simulink model "ac1_op_unlinked_R2016a"  (R2016a)
settings: Solver=ode23tb  SolverMode=SingleTasking  StartTime=0.0  StopTime=5  RelTol=1e-4
InitFcn:
  | %% Sys Para
  | fsw=10e3;
  | Ts_Control=1/fsw;
  | Tscon=Ts_Control;
  | Ts_Power=Ts_Control/32;
undefined symbols (not defined in the file): L2, R1, Rd
libraries: powerlib x8, powerlib_meascontrol x5
Description:
  | Copyright 2008-2017 The MathWorks, Inc.
settings Model: ExtModeTrigMode=oneshot  ExtModeArmWhenConnect=off  ExtModeAutoUpdateStatusClock=off  Creator=MathWorks  LastModifiedBy=CXIE
settings DataIOCC: ExternalInput=[]  SaveFormat=Array  SignalLoggingSaveFormat=ModelDataLogs  SaveOutput=off  SaveTime=off  SignalLoggingName=sigsOut
settings OptimizationCC: BlockReduction=off  BooleanDataType=off  ExpressionDepthLimit=2147483647  InitFltsAndDblsToZero=on  EfficientMapNaN2IntZero=off
settings DebuggingCC: UnderspecifiedInitializationDetection=Classic  MergeDetectMultiDrivingBlocksExec=none  CheckExecutionContextPreStartOutputMsg=on  CheckExecutionContextRuntimeOutputMsg=on  SignalResolutionControl=TryResolveAllWithWarning  MultiTaskDSMMsg=warning  MultiTaskCondExecSysMsg=none  SigSpecEnsureSampleTimeMsg=none  FcnCallInpInsideContextMsg=EnableAllAsWarning  StateNameClashWarn=warning
settings HardwareCC: ProdBitPerPointer=32  ProdLargestAtomicFloat=None  ProdIntDivRoundTo=Undefined  ProdEndianess=Unspecified  ProdWordSize=32  ProdHWDeviceType=32-bit Generic  TargetUnknown=on
settings ModelReferenceCC: PropagateSignalLabelsOutOfModel=off
settings GRTTargetCC: CombineOutputUpdateFcns=off  GRTInterface=on
settings ConfigComp: CovSFcnEnable=off
settings SimscapeCC: SimscapeNormalizeSystem=off  SimscapeNominalValues={1, 'bar'; 1, 'cm^3/s'; 1, 'bar*kg/s'; 1, 'kJ/kg'; 1, 'kW'; }

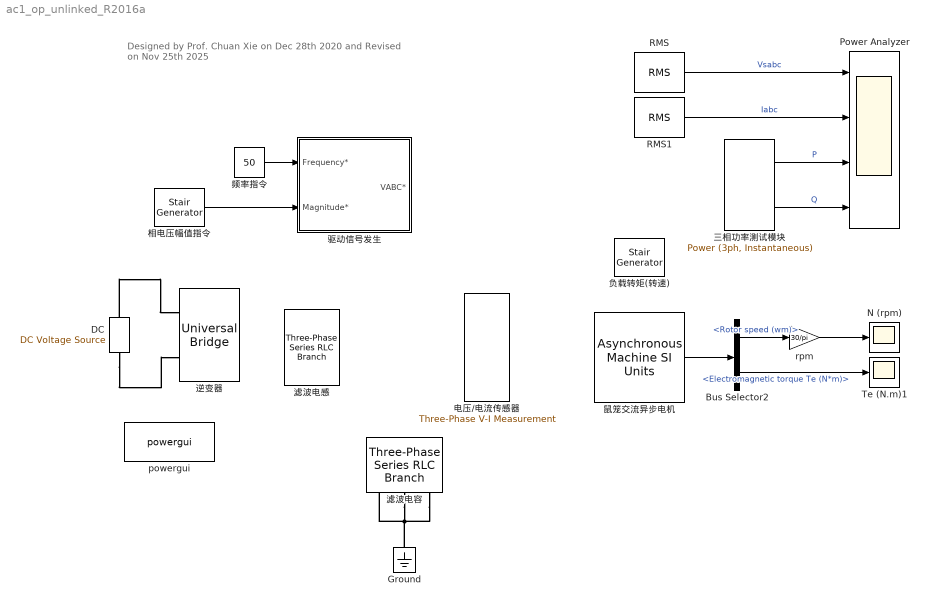
== system ac1_op_unlinked_R2016a ==
  note: Designed by Prof. Chuan Xie
      | on Dec 28th 2020
      | and Revised on Nov 25th 2025
  Bus Selector2 : BusSelector  OutputSignals=Mechanical.Rotor speed (wm),Mechanical.Electromagnetic torque Te (N*m)
  DC : powerlib/Electrical Sources/DC Voltage Source  Amplitude=650  Measurements=None
  Ground : powerlib/Elements/Ground  LConnTagsString=a
  N (rpm) : Scope
  Power Analyzer : Scope  NumInputPorts=4
  RMS : powerlib_meascontrol/Measurements/RMS  TrueRMS=on  Freq=50  RMSInit=120  Ts=0
  RMS1 : powerlib_meascontrol/Measurements/RMS  TrueRMS=on  Freq=50  RMSInit=120  Ts=0
  Te (N.m)1 : Scope
  powergui : powerlib/powergui  SimulationMode=Continuous  SampleTime=Ts_Power  frequency=60  Iterations=50  frequencyindice=50  Pbase=100e6  ErrMax=1e-4  UnitsV=kV  UnitsW=MW  buscounter=0  FunctionMessages=off  echomessages=off  EnableUseOfTLC=off  CurrentSourceSwitches=off  DisableSnubberDevices=off  DisableRonSwitches=off  DisableVfSwitches=off  DisplayEquations=off  AutomaticDiscreteSolvers=off  SolverType=Tustin  Interpol=off  ExternalGateDelay=off  methode=off  Ts=0  x0status=blocks  SPID=on  SwTol=0  HookPort=off  NonlinearTolerance=1e-4  nMaxIteration=100  ContinueOnMaxIteration=off  RestoreLinks=warning  ResistiveCurrentMeasurement=off  Frange=[0:2:500]  Ylog=off  Xlog=on  ShowGrid=off  save=off  variable=ZData  structure=0  ZoomFFT=on  StartTime=0.0  cycles=1  DisplayStyle=1  fundamental=60  FreqAxis=off  MaxFrequency=1000  frequencyindicesteady=1  RmsSteady=1  display=off
  rpm : Gain  Gain=30/pi  SaturateOnIntegerOverflow=on  OutDataTypeStr=Inherit: Same as input  ParamDataTypeStr=Inherit: Same as input
  三相功率测试模块 : powerlib_meascontrol/Measurements/Power (3ph, Instantaneous)
  滤波电容 : powerlib/Elements/Three-Phase Series RLC Branch  LConnTagsString=A|B|C  RConnTagsString=A|B|C  BranchType=C  Resistance=Rd  Inductance=L2  Capacitance=10e-6  Measurements=Branch currents
  滤波电感 : powerlib/Elements/Three-Phase Series RLC Branch  LConnTagsString=A|B|C  RConnTagsString=A|B|C  BranchType=L  Resistance=R1  Inductance=1e-3  Capacitance=1e-6  Measurements=Branch currents
  电压/电流传感器 : powerlib/Measurements/Three-Phase V-I Measurement  VoltageMeasurement=phase-to-ground  SetLabelV=off  LabelV=Vc1  Vpu=off  VpuLL=off  CurrentMeasurement=yes  SetLabelI=off  LabelI=IL1  Ipu=off  Pbase=100e6  Vbase=280  OutputType=Complex  PhasorSimulation=off  PSBequivalent=0
  相电压幅值指令 : powerlib_meascontrol/Pulse & Signal Generators/Stair Generator  t=[0]  e=[0]  Ts=0
  负载转矩(转速) : powerlib_meascontrol/Pulse & Signal Generators/Stair Generator  t=[0]  e=[0]  Ts=0
  逆变器 : powerlib/Power Electronics/Universal Bridge  Arms=3  SnubberResistance=1e5  SnubberCapacitance=inf  Device=Average-model based VSC  Ron=1e-3  Lon=0  ForwardVoltages="[  0  0  ]"  ForwardVoltage=0  GTOparameters=[ 10e-6 , 20e-6 ]  IGBTparameters=[ 1e-6 , 2e-6 ]  Measurements=None  Measurements_2=None  converterType=Rectifier
  频率指令 : Constant  Value=50
  驱动信号发生 : Subsystem
  鼠笼交流异步电机 : powerlib/Machines/Asynchronous Machine SI Units  RotorType=Squirrel-cage  PresetModel="17:  20 HP (15KW)   400 V 50Hz 1460 RPM"  MechanicalLoad=Mechanical rotational port  ShowDetailedParameters=on  ReferenceFrame=Rotor  Units=SI  MeasurementBus=off  NominalParameters=[1.5e+04 400 50]  Stator=[0.2147 0.000991]  Rotor=[0.2205 0.000991]  Cage1=[0.4155 0.002066]  Cage2=[0.4168 0.0003495]  Lm=0.06419  Mechanical=[0.102 0.009541 2]  PolePairs=2  InitialConditions="[ 1,0   0,0,0   0,0,0 ]"  SimulateSaturation=off  Saturation=[14.03593122, 27.81365428, 53.79336849, 72.68890987, 97.98006896, 148.6815601, 215.7428561, 302.9841135, 428.7778367 ; 230, 322, 414, 460, 506, 552, 598, 644, 690]  LoadFlowParameters=1492000  TsPowergui=0  TsBlock=-1  IterativeModel=Trapezoidal non iterative  IterativeDiscreteModel=Trapezoidal non iterative  Pmec=1.492e+006
  wires:
  rpm/1 -> N (rpm)/1
  Bus Selector2/2 -> Te (N.m)1/1  "<Electromagnetic torque Te (N*m)>"
  鼠笼交流异步电机/1 -> Bus Selector2/1
  Bus Selector2/1 -> rpm/1  "<Rotor speed (wm)>"
  频率指令/1 -> 驱动信号发生/1(Frequency*)
  相电压幅值指令/1 -> 驱动信号发生/2(Magnitude*)
  三相功率测试模块/2 -> Power Analyzer/4  "Q"
  三相功率测试模块/1 -> Power Analyzer/3  "P"
  RMS/1 -> Power Analyzer/1  "Vsabc"
  RMS1/1 -> Power Analyzer/2  "Iabc"
  connections:
  DC/RConn1 -- 逆变器/RConn1
  DC/LConn1 -- 逆变器/RConn2
  滤波电容/LConn2 -- Ground/LConn1 -- 滤波电容/LConn3 -- 滤波电容/LConn1

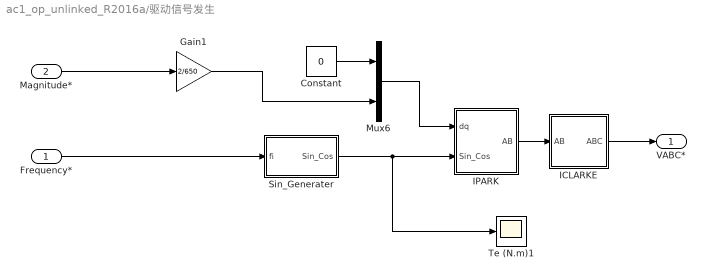
== system ac1_op_unlinked_R2016a/驱动信号发生 ==
  Frequency* : Inport
  Magnitude* : Inport  Port=2
  Constant : Constant  Value=0  SampleTime=Tscon
  Gain1 : Gain  Gain=2/650
  ICLARKE : Subsystem
  IPARK : Subsystem
  Mux6 : Mux  Inputs=2
  Sin_Generater : Subsystem
  Te (N.m)1 : Scope
  VABC* : Outport
  wires:
  Mux6/1 -> IPARK/1(dq)
  Magnitude*/1 -> Gain1/1
  Frequency*/1 -> Sin_Generater/1(fi)
  Sin_Generater/1(Sin_Cos) -> Te (N.m)1/1, IPARK/2(Sin_Cos)
  Constant/1 -> Mux6/1
  IPARK/1(AB) -> ICLARKE/1(AB)
  ICLARKE/1(ABC) -> VABC*/1
  Gain1/1 -> Mux6/2

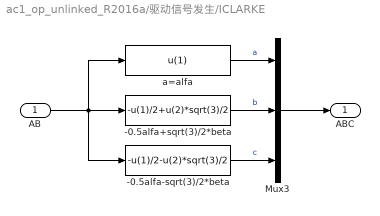
== system ac1_op_unlinked_R2016a/驱动信号发生/ICLARKE ==
  AB : Inport
  -0.5alfa+sqrt(3)/2*beta : Fcn  Expr=-u(1)/2+u(2)*sqrt(3)/2
  "-0.5alfa-sqrt(3)/2*beta " : Fcn  Expr=-u(1)/2-u(2)*sqrt(3)/2
  Mux3 : Mux  Inputs=3
  a=alfa : Fcn  Expr=u(1)
  ABC : Outport
  wires:
  -0.5alfa+sqrt(3)/2*beta/1 -> Mux3/2  "b"
  "-0.5alfa-sqrt(3)/2*beta "/1 -> Mux3/3  "c"
  Mux3/1 -> ABC/1
  AB/1 -> "-0.5alfa-sqrt(3)/2*beta "/1, -0.5alfa+sqrt(3)/2*beta/1, a=alfa/1
  a=alfa/1 -> Mux3/1  "a"

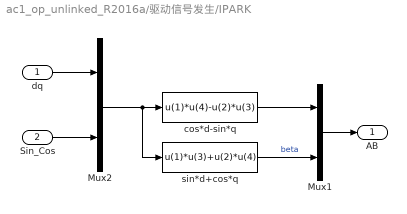
== system ac1_op_unlinked_R2016a/驱动信号发生/IPARK ==
  dq : Inport
  Sin_Cos : Inport  Port=2
  Mux1 : Mux  Inputs=2
  Mux2 : Mux  Inputs=2
  cos*d-sin*q : Fcn  Expr=u(1)*u(4)-u(2)*u(3)
  sin*d+cos*q : Fcn  Expr=u(1)*u(3)+u(2)*u(4)
  AB : Outport
  wires:
  Mux2/1 -> cos*d-sin*q/1, sin*d+cos*q/1
  Sin_Cos/1 -> Mux2/2
  dq/1 -> Mux2/1
  cos*d-sin*q/1 -> Mux1/1
  sin*d+cos*q/1 -> Mux1/2  "beta"
  Mux1/1 -> AB/1

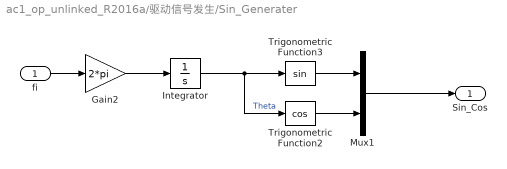
== system ac1_op_unlinked_R2016a/驱动信号发生/Sin_Generater ==
  fi : Inport
  Gain2 : Gain  Gain=2*pi
  Integrator : Integrator  WrapState=on  WrappedStateUpperValue=2*pi  WrappedStateLowerValue=0
  Mux1 : Mux  Inputs=[1 1]
  Trigonometric Function2 : Trigonometry  Operator=cos
  Trigonometric Function3 : Trigonometry
  Sin_Cos : Outport
  wires:
  Mux1/1 -> Sin_Cos/1
  Trigonometric Function3/1 -> Mux1/1
  Trigonometric Function2/1 -> Mux1/2
  fi/1 -> Gain2/1
  Gain2/1 -> Integrator/1
  Integrator/1 -> Trigonometric Function2/1, Trigonometric Function3/1  "Theta"
